simulink model "KUKA_simmechanic"  (R2015a)
settings: Solver=ode45  StartTime=0.0  StopTime=inf  RelTol=1e-3
undefined symbols (not defined in the file or in its folder): KUKA, part1, part2, part3, part4, RootGround, RootPart
libraries: mblibv1 x15
settings Model: Creator=PHANTU  LastModifiedBy=PHANTU
settings SimMechanicsCC: VisOnUpdateDiagram=on  VisDuringSimulation=on

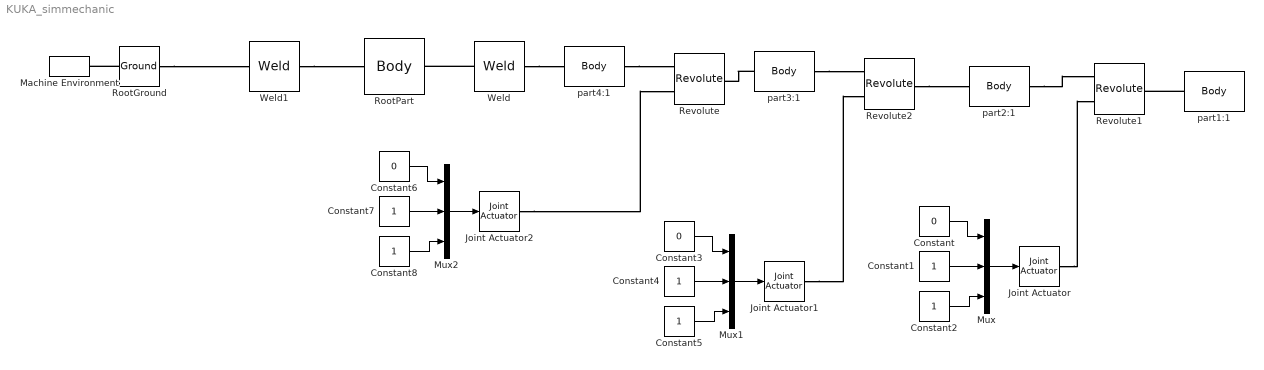
== system KUKA_simmechanic ==
  Constant : Constant  Value=0
  Constant{1..2,4..5,7..8} (6 alike) : Constant
  Constant3 : Constant  Value=0
  Constant6 : Constant  Value=0
  Joint Actuator : mblibv1/Sensors &  Actuators/Joint Actuator  UpdateFromCAD=off  PhysicalDomain=Mechanical  PortType=blob  ActuationStyle=Motion  AngleUnits=deg  ArcVelocityUnits=deg/s  ArcAccelerationUnits=deg/s^2  CoordPositionUnits=m  VelocityUnits=m/s  AccelerationUnits=m/s^2  ForceUnits=N  TorqueUnits=N*m  ActiveIO=on  Width=3  DialogClass=MechanicalActuatorBlock  Primitive=R1  ReferenceFrame=Absolute (World)
  Joint Actuator1 : mblibv1/Sensors &  Actuators/Joint Actuator  UpdateFromCAD=off  PhysicalDomain=Mechanical  PortType=blob  ActuationStyle=Motion  AngleUnits=deg  ArcVelocityUnits=deg/s  ArcAccelerationUnits=deg/s^2  CoordPositionUnits=m  VelocityUnits=m/s  AccelerationUnits=m/s^2  ForceUnits=N  TorqueUnits=N*m  ActiveIO=on  Width=3  DialogClass=MechanicalActuatorBlock  Primitive=R1  ReferenceFrame=Absolute (World)
  Joint Actuator2 : mblibv1/Sensors &  Actuators/Joint Actuator  UpdateFromCAD=off  PhysicalDomain=Mechanical  PortType=blob  ActuationStyle=Motion  AngleUnits=deg  ArcVelocityUnits=deg/s  ArcAccelerationUnits=deg/s^2  CoordPositionUnits=m  VelocityUnits=m/s  AccelerationUnits=m/s^2  ForceUnits=N  TorqueUnits=N*m  ActiveIO=on  Width=3  DialogClass=MechanicalActuatorBlock  Primitive=R1  ReferenceFrame=Absolute (World)
  Machine Environment : mblibv1/Bodies/Machine Environment  PortType=env  PhysicalDomain=Mechanical  DialogTemplateClass=MECH.MachineEnvironment  SyncWhenCopied=off  Gravity=[0 -9.81 0]  GravityUnits=m/s^2  GravityAsSignal=off  Dimensionality=Auto-detect  AnalysisType=Forward dynamics  LinearAssemblyTolerance=1e-3  LinearAssemblyToleranceUnits=m  AngularAssemblyTolerance=1e-3  AngularAssemblyToleranceUnits=rad  ConstraintSolverType=Stabilizing  ConstraintRelTolerance=1e-4  ConstraintAbsTolerance=1e-4  UseRobustSingularityHandling=off  RedundancyAnalysisToleranceType=Automatically select tolerance  RedundancyAnalysisTolerance=1e-14  StatePerturbationType=Fixed  PerturbationSize=1e-5  VisualizeMachine=on  BodyVisualizationType=Use model default body geometries  BodyColorSelMode=Use model default  DefaultBodyColor=[1 0 0]
  Mux : Mux  Inputs=3
  Mux1 : Mux  Inputs=3
  Mux2 : Mux  Inputs=3
  Revolute : mblibv1/Joints/Revolute  LConnTagsString=__newl0|SA1  RConnTagsString=__newr0  UpdateFromCAD=on  PMImportedID=part3:1:-:part4:1  NumSAPorts=1  CutJoint=off  MarkAsCut=off  Primitives=prismatic  PrimitiveProps=R1$World$[0,0,-1]$revolute  DialogClass=JointBlock  R1Axis=[0,0,-1]
  Revolute1 : mblibv1/Joints/Revolute  LConnTagsString=__newl0|SA1  RConnTagsString=__newr0  UpdateFromCAD=on  PMImportedID=part1:1:-:part2:1  NumSAPorts=1  CutJoint=off  MarkAsCut=off  Primitives=prismatic  PrimitiveProps=R1$World$[0,-1,0]$revolute  DialogClass=JointBlock  R1Axis=[0,-1,0]
  Revolute2 : mblibv1/Joints/Revolute  LConnTagsString=__newl0|SA1  RConnTagsString=__newr0  UpdateFromCAD=on  PMImportedID=part2:1:-:part3:1  NumSAPorts=1  CutJoint=off  MarkAsCut=off  Primitives=prismatic  PrimitiveProps=R1$World$[0,-1,0]$revolute  DialogClass=JointBlock  R1Axis=[0,-1,0]
  RootGround : mblibv1/Bodies/Ground  UpdateFromCAD=on  PMImportedID=RootGround  LeftPortType=env  RightPortType=workingframe  PhysicalDomain=Mechanical  DialogClass=GroundBlock  CoordPosition=[114.791,-2.42393,693.337]  CoordPositionUnits=mm  StateVectorMgrId=0  MachineId=[1 0]  ShowEnvPort=on  ParameterChecksum=[1042391727, 4180609376, 1395604701, 2490994427]  TopologyChecksum=[2657798021, 3534535307, 3409893197, 2609067154]
  RootPart : mblibv1/Bodies/Body  LConnTagsString=CS3  RConnTagsString=CS2  UpdateFromCAD=on  PMImportedID=KUKA/RootPart  DialogClass=MechanicalBodyBlock  Mass=0  MassUnits=kg  InertiaUnits=kg*m^2  Inertia=[0,0,0;0,0,0;0,0,0]  Shape=Cylinder  ShapeDims=[1 1]  ShapeUnits=m  ShapeUse=false  Density=1  DensityUnits=kg/m^3  DensityUse=false  GraphicsMode=MACHINE_DEFAULT  BodyColorSelMode=MACHINE_DEFAULT  BodyColor=[1 0 0]  AttachedToCS=CS1  CG=Right$CG$[114.791 -2.42393 693.337]$WORLD$WORLD$mm$[1 0 0;0 1 0;0 0 1]$3x3 Transform$rad$WORLD$false$KUKA/RootPart::CG(AUTOGEN)  WorkingFrames=Right$CS1$[0 0 0]$WORLD$WORLD$mm$[1 0 0;0 1 0;0 0 1]$3x3 Transform$rad$WORLD$false$KUKA/RootPart::CS1(AUTOGEN)#Right$CS2$[-41.1494 -3.79313 230.033]$WORLD$WORLD$mm$[1 0 0;0 1 0;0 0 1]$3x3 Transform$rad$WORLD$true$:-:part4:1::KUKA/RootPart(AUTOGEN)#Left$CS3$[114.791 -2.42393 693.337]$WORLD$WORLD$mm$[1 0 0;0 1 0;0 0 1]$3x3 Transform$rad$WORLD$true$KUKA/RootPart:-:RootGround::KUKA/RootPart(AUTOGEN)  CGPos=[114.791 -2.42393 693.337]  CGRot=[1 0 0;0 1 0;0 0 1]  CS0Pos=[]  CS0Rot=[]  CS1Pos=[0 0 0]  CS1Rot=[1 0 0;0 1 0;0 0 1]  CS2Pos=[-41.1494 -3.79313 230.033]  CS2Rot=[1 0 0;0 1 0;0 0 1]  CS3Pos=[114.791 -2.42393 693.337]  CS3Rot=[1 0 0;0 1 0;0 0 1]  CS4Pos=[]  CS4Rot=[]  CS5Pos=[]  CS5Rot=[]  CS6Pos=[]  CS6Rot=[]  CS7Pos=[]  CS7Rot=[]  CS8Pos=[]  CS8Rot=[]  CS9Pos=[]  CS9Rot=[]  CS10Pos=[]  CS10Rot=[]  CS11Pos=[]  CS11Rot=[]  CS12Pos=[]  CS12Rot=[]  CS13Pos=[]  CS13Rot=[]  CS14Pos=[]  CS14Rot=[]  CS15Pos=[]  CS15Rot=[]  CS16Pos=[]  CS16Rot=[]  CS17Pos=[]  CS17Rot=[]  CS18Pos=[]  CS18Rot=[]  CS19Pos=[]  CS19Rot=[]  CS20Pos=[]  CS20Rot=[]
  Weld : mblibv1/Joints/Weld  LConnTagsString=__newl0  RConnTagsString=__newr0  UpdateFromCAD=on  PMImportedID=:-:part4:1  NumSAPorts=0  CutJoint=off  MarkAsCut=off  Primitives=weld  PrimitiveProps=W$WORLD$[0.57735,0.57735,0.57735]$weld  DialogClass=JointBlock  WAxis=[0.57735,0.57735,0.57735]
  Weld1 : mblibv1/Joints/Weld  LConnTagsString=__newl0  RConnTagsString=__newr0  UpdateFromCAD=on  PMImportedID=KUKA/RootPart:-:RootGround  NumSAPorts=0  CutJoint=off  MarkAsCut=off  Primitives=weld  PrimitiveProps=W$WORLD$[0.57735,0.57735,0.57735]$weld  DialogClass=JointBlock  WAxis=[0.57735,0.57735,0.57735]
  part1:1 : mblibv1/Bodies/Body  LConnTagsString=CS2  RConnTagsString=CS3  UpdateFromCAD=on  PMImportedID=part1:1  DialogClass=MechanicalBodyBlock  Mass=40.4989  MassUnits=kg  InertiaUnits=kg*m^2  Inertia=[0.772378,0.243082,0.407747;0.243082,3.65301,-0.170622;0.407747,-0.170622,3.50439]  Shape=Cylinder  ShapeDims=[1 1]  ShapeUnits=m  ShapeUse=false  Density=1  DensityUnits=kg/m^3  DensityUse=false  GraphicsMode=GFXFILE  GraphicsFileName=part1_ipt_86567821.STL  BodyColorSelMode=COLORPALETTE  BodyColor=[0.74902 0.74902 0.74902]  AttachedToCS=CS1  CG=Right$CG$[337.651 45.7629 1451.73]$WORLD$WORLD$mm$[1 0 0;0 1 0;0 0 1]$3x3 Transform$rad$WORLD$false$part1:1::CG(AUTOGEN)  WorkingFrames=Right$CS1$[0 0 31.6765]$WORLD$WORLD$mm$[1 0 0;0 1 0;0 0 1]$3x3 Transform$rad$WORLD$false$part1:1::CS1(AUTOGEN)#Left$CS2$[260 -107 1386.68]$WORLD$WORLD$mm$[1 0 0;0 1 0;0 0 1]$3x3 Transform$rad$WORLD$true$part1:1:-:part2:1::part1:1(AUTOGEN)#Right$CS3$[1082 0 1351]$WORLD$WORLD$mm$[1 0 0;0 1 0;0 0 1]$3x3 Transform$rad$WORLD$true$none  CGPos=[337.651 45.7629 1451.73]  CGRot=[1 0 0;0 1 0;0 0 1]  CS0Pos=[]  CS0Rot=[]  CS1Pos=[0 0 31.6765]  CS1Rot=[1 0 0;0 1 0;0 0 1]  CS2Pos=[260 -107 1386.68]  CS2Rot=[1 0 0;0 1 0;0 0 1]  CS3Pos=[1082 0 1351]  CS3Rot=[1 0 0;0 1 0;0 0 1]  CS4Pos=[]  CS4Rot=[]  CS5Pos=[]  CS5Rot=[]  CS6Pos=[]  CS6Rot=[]  CS7Pos=[]  CS7Rot=[]  CS8Pos=[]  CS8Rot=[]  CS9Pos=[]  CS9Rot=[]  CS10Pos=[]  CS10Rot=[]  CS11Pos=[]  CS11Rot=[]  CS12Pos=[]  CS12Rot=[]  CS13Pos=[]  CS13Rot=[]  CS14Pos=[]  CS14Rot=[]  CS15Pos=[]  CS15Rot=[]  CS16Pos=[]  CS16Rot=[]  CS17Pos=[]  CS17Rot=[]  CS18Pos=[]  CS18Rot=[]  CS19Pos=[]  CS19Rot=[]  CS20Pos=[]  CS20Rot=[]
  part2:1 : mblibv1/Bodies/Body  LConnTagsString=CS3  RConnTagsString=CS2  UpdateFromCAD=on  PMImportedID=part2:1  DialogClass=MechanicalBodyBlock  Mass=13.5189  MassUnits=kg  InertiaUnits=kg*m^2  Inertia=[0.595755,-0.000241052,-0.000341583;-0.000241052,0.593927,0.0264066;-0.000341583,0.0264066,0.0592214]  Shape=Cylinder  ShapeDims=[1 1]  ShapeUnits=m  ShapeUse=false  Density=1  DensityUnits=kg/m^3  DensityUse=false  GraphicsMode=GFXFILE  GraphicsFileName=part2_ipt_86567821.STL  BodyColorSelMode=COLORPALETTE  BodyColor=[0.74902 0.74902 0.74902]  AttachedToCS=CS1  CG=Right$CG$[260.236 -180.551 1028.07]$WORLD$WORLD$mm$[1 0 0;0 1 0;0 0 1]$3x3 Transform$rad$WORLD$false$part2:1::CG(AUTOGEN)  WorkingFrames=Right$CS1$[0 0 31.6765]$WORLD$WORLD$mm$[1 0 0;0 1 0;0 0 1]$3x3 Transform$rad$WORLD$false$part2:1::CS1(AUTOGEN)#Right$CS2$[260 -107 1386.68]$WORLD$WORLD$mm$[1 0 0;0 1 0;0 0 1]$3x3 Transform$rad$WORLD$true$part1:1:-:part2:1::part2:1(AUTOGEN)#Left$CS3$[260 -83 706.677]$WORLD$WORLD$mm$[1 0 0;0 1 0;0 0 1]$3x3 Transform$rad$WORLD$true$part2:1:-:part3:1::part2:1(AUTOGEN)  CGPos=[260.236 -180.551 1028.07]  CGRot=[1 0 0;0 1 0;0 0 1]  CS0Pos=[]  CS0Rot=[]  CS1Pos=[0 0 31.6765]  CS1Rot=[1 0 0;0 1 0;0 0 1]  CS2Pos=[260 -107 1386.68]  CS2Rot=[1 0 0;0 1 0;0 0 1]  CS3Pos=[260 -83 706.677]  CS3Rot=[1 0 0;0 1 0;0 0 1]  CS4Pos=[]  CS4Rot=[]  CS5Pos=[]  CS5Rot=[]  CS6Pos=[]  CS6Rot=[]  CS7Pos=[]  CS7Rot=[]  CS8Pos=[]  CS8Rot=[]  CS9Pos=[]  CS9Rot=[]  CS10Pos=[]  CS10Rot=[]  CS11Pos=[]  CS11Rot=[]  CS12Pos=[]  CS12Rot=[]  CS13Pos=[]  CS13Rot=[]  CS14Pos=[]  CS14Rot=[]  CS15Pos=[]  CS15Rot=[]  CS16Pos=[]  CS16Rot=[]  CS17Pos=[]  CS17Rot=[]  CS18Pos=[]  CS18Rot=[]  CS19Pos=[]  CS19Rot=[]  CS20Pos=[]  CS20Rot=[]
  part3:1 : mblibv1/Bodies/Body  LConnTagsString=CS2  RConnTagsString=CS3  UpdateFromCAD=on  PMImportedID=part3:1  DialogClass=MechanicalBodyBlock  Mass=28.3532  MassUnits=kg  InertiaUnits=kg*m^2  Inertia=[1.07185,-0.0539717,-0.354129;-0.0539717,1.05703,-0.0608066;-0.354129,-0.0608066,1.30191]  Shape=Cylinder  ShapeDims=[1 1]  ShapeUnits=m  ShapeUse=false  Density=1  DensityUnits=kg/m^3  DensityUse=false  GraphicsMode=GFXFILE  GraphicsFileName=part3_ipt_86567821.STL  BodyColorSelMode=COLORPALETTE  BodyColor=[0.74902 0.74902 0.74902]  AttachedToCS=CS1  CG=Right$CG$[107.444 17.0185 580.451]$WORLD$WORLD$mm$[1 0 0;0 1 0;0 0 1]$3x3 Transform$rad$WORLD$false$part3:1::CG(AUTOGEN)  WorkingFrames=Right$CS1$[0 0 31.6765]$WORLD$WORLD$mm$[1 0 0;0 1 0;0 0 1]$3x3 Transform$rad$WORLD$false$part3:1::CS1(AUTOGEN)#Left$CS2$[0 0 428.6]$WORLD$WORLD$mm$[1 0 0;0 1 0;0 0 1]$3x3 Transform$rad$WORLD$true$part3:1:-:part4:1::part3:1(AUTOGEN)#Right$CS3$[260 -83 706.677]$WORLD$WORLD$mm$[1 0 0;0 1 0;0 0 1]$3x3 Transform$rad$WORLD$true$part2:1:-:part3:1::part3:1(AUTOGEN)  CGPos=[107.444 17.0185 580.451]  CGRot=[1 0 0;0 1 0;0 0 1]  CS0Pos=[]  CS0Rot=[]  CS1Pos=[0 0 31.6765]  CS1Rot=[1 0 0;0 1 0;0 0 1]  CS2Pos=[0 0 428.6]  CS2Rot=[1 0 0;0 1 0;0 0 1]  CS3Pos=[260 -83 706.677]  CS3Rot=[1 0 0;0 1 0;0 0 1]  CS4Pos=[]  CS4Rot=[]  CS5Pos=[]  CS5Rot=[]  CS6Pos=[]  CS6Rot=[]  CS7Pos=[]  CS7Rot=[]  CS8Pos=[]  CS8Rot=[]  CS9Pos=[]  CS9Rot=[]  CS10Pos=[]  CS10Rot=[]  CS11Pos=[]  CS11Rot=[]  CS12Pos=[]  CS12Rot=[]  CS13Pos=[]  CS13Rot=[]  CS14Pos=[]  CS14Rot=[]  CS15Pos=[]  CS15Rot=[]  CS16Pos=[]  CS16Rot=[]  CS17Pos=[]  CS17Rot=[]  CS18Pos=[]  CS18Rot=[]  CS19Pos=[]  CS19Rot=[]  CS20Pos=[]  CS20Rot=[]
  part4:1 : mblibv1/Bodies/Body  LConnTagsString=CS2  RConnTagsString=CS3  UpdateFromCAD=on  PMImportedID=part4:1  DialogClass=MechanicalBodyBlock  Mass=69.1518  MassUnits=kg  InertiaUnits=kg*m^2  Inertia=[1.73395,-0.0485512,-0.0688783;-0.0485512,2.09396,-0.000359291;-0.0688783,-0.000359291,2.19578]  Shape=Cylinder  ShapeDims=[1 1]  ShapeUnits=m  ShapeUse=false  Density=1  DensityUnits=kg/m^3  DensityUse=false  GraphicsMode=GFXFILE  GraphicsFileName=part4_ipt_86567821.STL  BodyColorSelMode=COLORPALETTE  BodyColor=[0.74902 0.74902 0.74902]  AttachedToCS=CS1  CG=Right$CG$[-41.1494 -3.79313 230.033]$WORLD$WORLD$mm$[1 0 0;0 1 0;0 0 1]$3x3 Transform$rad$WORLD$false$part4:1::CG(AUTOGEN)  WorkingFrames=Right$CS1$[0.557964 0.1152 30]$WORLD$WORLD$mm$[1 0 0;0 1 0;0 0 1]$3x3 Transform$rad$WORLD$false$part4:1::CS1(AUTOGEN)#Left$CS2$[-41.1494 -3.79313 230.033]$WORLD$WORLD$mm$[1 0 0;0 1 0;0 0 1]$3x3 Transform$rad$WORLD$true$:-:part4:1::part4:1(AUTOGEN)#Right$CS3$[0 0 428.6]$WORLD$WORLD$mm$[1 0 0;0 1 0;0 0 1]$3x3 Transform$rad$WORLD$true$part3:1:-:part4:1::part4:1(AUTOGEN)  CGPos=[-41.1494 -3.79313 230.033]  CGRot=[1 0 0;0 1 0;0 0 1]  CS0Pos=[]  CS0Rot=[]  CS1Pos=[0.557964 0.1152 30]  CS1Rot=[1 0 0;0 1 0;0 0 1]  CS2Pos=[-41.1494 -3.79313 230.033]  CS2Rot=[1 0 0;0 1 0;0 0 1]  CS3Pos=[0 0 428.6]  CS3Rot=[1 0 0;0 1 0;0 0 1]  CS4Pos=[]  CS4Rot=[]  CS5Pos=[]  CS5Rot=[]  CS6Pos=[]  CS6Rot=[]  CS7Pos=[]  CS7Rot=[]  CS8Pos=[]  CS8Rot=[]  CS9Pos=[]  CS9Rot=[]  CS10Pos=[]  CS10Rot=[]  CS11Pos=[]  CS11Rot=[]  CS12Pos=[]  CS12Rot=[]  CS13Pos=[]  CS13Rot=[]  CS14Pos=[]  CS14Rot=[]  CS15Pos=[]  CS15Rot=[]  CS16Pos=[]  CS16Rot=[]  CS17Pos=[]  CS17Rot=[]  CS18Pos=[]  CS18Rot=[]  CS19Pos=[]  CS19Rot=[]  CS20Pos=[]  CS20Rot=[]
  wires:
  Mux/1 -> Joint Actuator/1
  Constant/1 -> Mux/1
  Constant1/1 -> Mux/2
  Constant2/1 -> Mux/3
  Mux1/1 -> Joint Actuator1/1
  Constant3/1 -> Mux1/1
  Constant4/1 -> Mux1/2
  Constant5/1 -> Mux1/3
  Mux2/1 -> Joint Actuator2/1
  Constant6/1 -> Mux2/1
  Constant7/1 -> Mux2/2
  Constant8/1 -> Mux2/3
  connections:
  RootGround/RConn1 -- Weld1/LConn1
  Weld1/RConn1 -- RootPart/LConn1
  RootGround/LConn1 -- Machine Environment/RConn1
  Joint Actuator/RConn1 -- Revolute1/LConn2
  Joint Actuator1/RConn1 -- Revolute2/LConn2
  Joint Actuator2/RConn1 -- Revolute/LConn2
  Weld/LConn1 -- RootPart/RConn1
  Weld/RConn1 -- part4:1/LConn1
  part4:1/RConn1 -- Revolute/LConn1
  part3:1/LConn1 -- Revolute/RConn1
  part3:1/RConn1 -- Revolute2/LConn1
  Revolute2/RConn1 -- part2:1/LConn1
  part2:1/RConn1 -- Revolute1/LConn1
  part1:1/LConn1 -- Revolute1/RConn1
